simulink model "DualBuckPPS22016"  (R2024b)
settings: Solver=ode45  StartTime=0.0  StopTime=0.5  RelTol=1e-3
model workspace (MAT data in the model file):
  D = 50
  T = 0.0333333333333
undefined symbols (not defined in the file): D_T_DOWN_Given, D_T_UP_Given, DiscIntNeverNeededParam, P, T_pulse, TP
libraries: spsOnDelayLib x30, dspsnks4 x12, dspfdesign x11, spsCurrentMeasurementLib x11, spsSeriesRLCBranchLib x6, spsMosfetLib x4, slpidlib x4, spsVoltageMeasurementLib x4, simulink x3, spsControlledCurrentSourceLib x1, spsDCVoltageSourceLib x1, spspowerguiLib x1
(part 2 of 2)

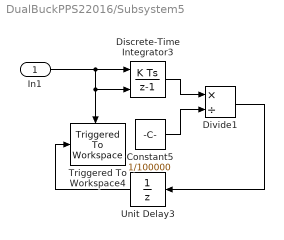
== system DualBuckPPS22016/Subsystem5 ==
  In1 : Inport
  Constant5 : Constant  Value=1/100000
  Discrete-Time Integrator3 : DiscreteIntegrator  ExternalReset=falling  SampleTime=-1  ICPrevOutput=DiscIntNeverNeededParam  ICPrevScaledInput=DiscIntNeverNeededParam
  Divide1 : Product  Inputs=*/
  Triggered To Workspace4 : dspsnks4/Triggered To Workspace  TriggerType=Falling edge  VariableName=PWM_S_DOWN  Buffer=1000  Save2DMode=2-D array (concatenate along first dimension)
      settings: FixptAsFi=off
  Unit Delay3 : UnitDelay  SampleTime=-1  HasFrameUpgradeWarning=on
  wires:
  Unit Delay3/1 -> Triggered To Workspace4/1
  Discrete-Time Integrator3/1 -> Divide1/1
  Constant5/1 -> Divide1/2
  Divide1/1 -> Unit Delay3/1
  In1/1 -> Discrete-Time Integrator3/1, Triggered To Workspace4/Trigger, Discrete-Time Integrator3/2

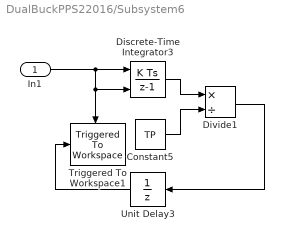
== system DualBuckPPS22016/Subsystem6 ==
  In1 : Inport
  Constant5 : Constant  Value=TP
  Discrete-Time Integrator3 : DiscreteIntegrator  ExternalReset=falling  SampleTime=-1  ICPrevOutput=DiscIntNeverNeededParam  ICPrevScaledInput=DiscIntNeverNeededParam
  Divide1 : Product  Inputs=*/
  Triggered To Workspace1 : dspsnks4/Triggered To Workspace  TriggerType=Falling edge  VariableName=VC1_DOWN  Buffer=1000  Save2DMode=2-D array (concatenate along first dimension)
      settings: FixptAsFi=off
  Unit Delay3 : UnitDelay  SampleTime=-1  HasFrameUpgradeWarning=on
  wires:
  Unit Delay3/1 -> Triggered To Workspace1/1
  Discrete-Time Integrator3/1 -> Divide1/1
  In1/1 -> Discrete-Time Integrator3/1, Discrete-Time Integrator3/2, Triggered To Workspace1/Trigger
  Constant5/1 -> Divide1/2
  Divide1/1 -> Unit Delay3/1

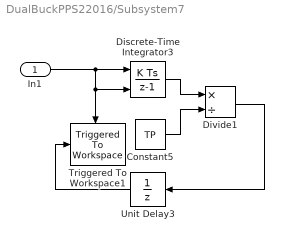
== system DualBuckPPS22016/Subsystem7 ==
  In1 : Inport
  Constant5 : Constant  Value=TP
  Discrete-Time Integrator3 : DiscreteIntegrator  ExternalReset=falling  SampleTime=-1  ICPrevOutput=DiscIntNeverNeededParam  ICPrevScaledInput=DiscIntNeverNeededParam
  Divide1 : Product  Inputs=*/
  Triggered To Workspace1 : dspsnks4/Triggered To Workspace  TriggerType=Falling edge  VariableName=VG1_UP  Buffer=1000  Save2DMode=2-D array (concatenate along first dimension)
      settings: FixptAsFi=off
  Unit Delay3 : UnitDelay  SampleTime=-1  HasFrameUpgradeWarning=on
  wires:
  Unit Delay3/1 -> Triggered To Workspace1/1
  Discrete-Time Integrator3/1 -> Divide1/1
  In1/1 -> Discrete-Time Integrator3/1, Discrete-Time Integrator3/2, Triggered To Workspace1/Trigger
  Constant5/1 -> Divide1/2
  Divide1/1 -> Unit Delay3/1

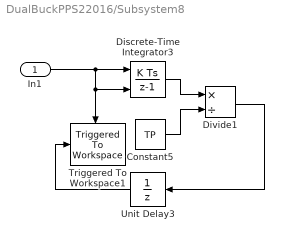
== system DualBuckPPS22016/Subsystem8 ==
  In1 : Inport
  Constant5 : Constant  Value=TP
  Discrete-Time Integrator3 : DiscreteIntegrator  ExternalReset=falling  SampleTime=-1  ICPrevOutput=DiscIntNeverNeededParam  ICPrevScaledInput=DiscIntNeverNeededParam
  Divide1 : Product  Inputs=*/
  Triggered To Workspace1 : dspsnks4/Triggered To Workspace  TriggerType=Falling edge  VariableName=VG1_DOWN  Buffer=1000  Save2DMode=2-D array (concatenate along first dimension)
      settings: FixptAsFi=off
  Unit Delay3 : UnitDelay  SampleTime=-1  HasFrameUpgradeWarning=on
  wires:
  Divide1/1 -> Unit Delay3/1
  Constant5/1 -> Divide1/2
  In1/1 -> Triggered To Workspace1/Trigger, Discrete-Time Integrator3/2, Discrete-Time Integrator3/1
  Discrete-Time Integrator3/1 -> Divide1/1
  Unit Delay3/1 -> Triggered To Workspace1/1

== system DualBuckPPS22016/Subsystem9 ==
  In : Inport
  On Delay10 : spsOnDelayLib/On Delay  DelayType=On delay  delay=10e-6  ic=0  Ts=0
  On Delay11 : spsOnDelayLib/On Delay  DelayType=Off delay  delay=ceil(TP*1e5)*1e-5-TP  ic=0  Ts=0
  Out : Outport
  wires:
  On Delay10/1 -> On Delay11/1
  In/1 -> On Delay10/1
  On Delay11/1 -> Out/1

== system DualBuckPPS22016/Triggered Subsystem ==
  In1 : Inport
  Trigger : TriggerPort  VariantControl=(inherit)
  Out1 : Outport
  wires:
  In1/1 -> Out1/1

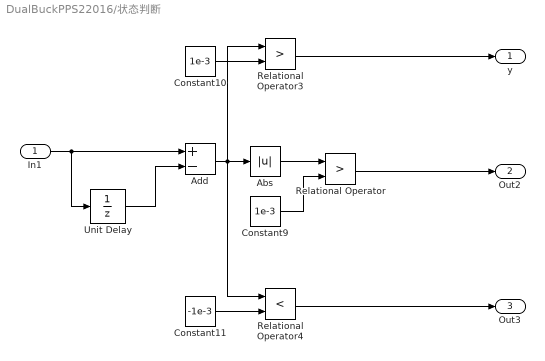
== system DualBuckPPS22016/状态判断 ==
  In1 : Inport
  Abs : Abs  SaturateOnIntegerOverflow=off
  Add : Sum  Inputs=+-
  Constant10 : Constant  Value=1e-3
  Constant11 : Constant  Value=-1e-3
  Constant9 : Constant  Value=1e-3
  Relational Operator : RelationalOperator  Operator=>  OutDataTypeStr=boolean  RndMeth=Simplest  InputSameDT=off
  Relational Operator3 : RelationalOperator  Operator=>  OutDataTypeStr=boolean  RndMeth=Simplest  InputSameDT=off
  Relational Operator4 : RelationalOperator  Operator=<  OutDataTypeStr=boolean  RndMeth=Simplest  InputSameDT=off
  Unit Delay : UnitDelay  SampleTime=-1  HasFrameUpgradeWarning=on
  y : Outport
  Out2 : Outport  Port=2
  Out3 : Outport  Port=3
  wires:
  In1/1 -> Unit Delay/1, Add/1
  Constant10/1 -> Relational Operator3/2
  Unit Delay/1 -> Add/2
  Constant9/1 -> Relational Operator/2
  Constant11/1 -> Relational Operator4/2
  Add/1 -> Relational Operator4/1, Relational Operator3/1, Abs/1
  Abs/1 -> Relational Operator/1
  Relational Operator3/1 -> y/1
  Relational Operator/1 -> Out2/1
  Relational Operator4/1 -> Out3/1

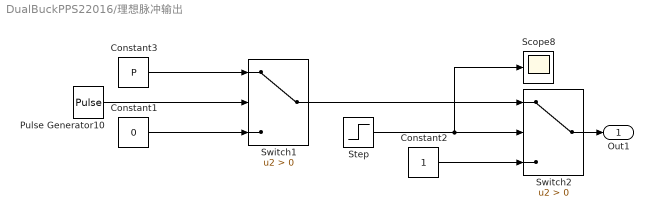
== system DualBuckPPS22016/理想脉冲输出 ==
  Constant1 : Constant  Value=0
  Constant2 : Constant
  Constant3 : Constant  Value=P
  Pulse Generator10 : DiscretePulseGenerator  PulseType=Time based  Period=T  PulseWidth=D  VectorParams1D=off
  Scope8 : Scope
  Step : Step  Time=0  SampleTime=0
  Switch1 : Switch  Criteria=u2 > Threshold  SaturateOnIntegerOverflow=off  InputSameDT=off
  Switch2 : Switch  Criteria=u2 > Threshold  SaturateOnIntegerOverflow=off  InputSameDT=off
  Out1 : Outport
  wires:
  Switch2/1 -> Out1/1
  Constant1/1 -> Switch1/3
  Step/1 -> Scope8/1, Switch2/2
  Switch1/1 -> Switch2/1
  Pulse Generator10/1 -> Switch1/2
  Constant2/1 -> Switch2/3
  Constant3/1 -> Switch1/1

== matlab function DualBuckPPS22016/MATLAB Function4 ==
  data: Q_main output; Q_sync output; Vref input; Vo input; Iref_ext input; iL input; voltage_PI_out output; current_error output; T_period output
function [Q_main, Q_sync, voltage_PI_out, ...
          current_error, T_period] = ...
    Buck_Double_COT(Vref, Vo, Iref_ext, iL)
%#codegen
%
% 单路同步Buck：
% 电压外环PI + 电流比较型COT控制
%
% 输入：
% Vref     ：输出电压参考值
% Vo       ：实际输出电压
% Iref_ext ：外部电感电流参考值
% iL       ：实际电感电流
%
% 输出：
% Q_main         ：主开关驱动信号
% Q_sync         ：同步开关驱动信号
% voltage_PI_out ：电压外环PI输出
% current_error  ：电流比较误差
% T_period       ：最近一个完整COT开关周期，单位为s
%
% 电流误差保持原有定义：
%
% current_error = voltage_PI_out - Iref_ext - iL
%
% 当current_error >= I_trigger，
% 并且满足最小关断时间时，
% 主开关固定导通Ton。

%% ===================== 1. 控制参数 =====================

Ts = 100e-9;                       % MATLAB Function执行周期

Kpv = 0.02;                        % 电压外环比例系数

Kiv = 0.2;                         % 电压外环积分系数

Ton = 2e-6;                        % COT固定导通时间

Toff_min = Ts;                     % 两个脉冲之间的最小关断时间

I_trigger = 0.2;                   % COT电流误差触发阈值

N_on = max(1, round(Ton / Ts));    % 固定导通时间对应的采样点数

N_off = max(1, round(Toff_min / Ts));
                                      % 最小关断时间对应的采样点数

%% ===================== 2. 持久变量 =====================

persistent voltage_integral        % 电压PI积分项

persistent on_count                % 固定导通剩余采样点数

persistent off_count               % 当前连续关断采样点数

persistent period_count            % 当前开关周期采样点计数

persistent last_period_count       % 最近一个完整开关周期采样点数

persistent first_pulse_generated   % 是否已经产生过第一个脉冲

%% ===================== 3. 第一次运行初始化 =====================

if isempty(voltage_integral)

    voltage_integral = 0.0;         % PI积分项初始化

    on_count = 0.0;                 % 初始不处于固定导通阶段

    off_count = N_off;              % 初始允许产生第一个脉冲

    period_count = 0.0;             % 当前周期计数初始化

    last_period_count = 0.0;        % 尚未测得完整周期

    first_pulse_generated = false;  % 尚未产生第一个脉冲

end

%% ===================== 4. 电压外环PI =====================

voltage_error = Vref - Vo;          % 计算输出电压误差

voltage_integral = voltage_integral ...
                 + Kiv * voltage_error * Ts;
                                      % 更新电压PI积分项

voltage_PI_out = Kpv * voltage_error ...
               + voltage_integral;
                                      % 计算电压PI输出

%% ===================== 5. 电流比较与触发请求 =====================

current_error = voltage_PI_out ...
              - Iref_ext ...
              - iL;
                                      % 保持原有电流误差逻辑

cot_request = current_error >= I_trigger;
                                      % 判断是否满足COT触发条件

%% ===================== 6. 开关周期计数 =====================

period_count = period_count + 1.0;  % 统计两次脉冲起点之间的采样点数

%% ===================== 7. 默认主开关状态 =====================

Q_main = false;                     % 默认主开关关断

%% ===================== 8. COT固定导通阶段 =====================

if on_count > 0.0

    Q_main = true;                  % 固定导通时间内保持主开关导通

    on_count = on_count - 1.0;      % 固定导通剩余计数减1

    if on_count <= 0.0

        on_count = 0.0;             % 固定导通时间结束

        off_count = 0.0;            % 开始统计最小关断时间

    end

%% ===================== 9. COT关断等待阶段 =====================

else

    if cot_request && (off_count >= N_off)

        % 第一次脉冲没有前一个脉冲，因此不能计算完整周期
        if first_pulse_generated

            last_period_count = max(1.0, period_count);
                                      % 保存本次脉冲与上次脉冲之间的周期

        else

            first_pulse_generated = true;
                                      % 标记第一个脉冲已经产生

        end

        period_count = 0.0;         % 从当前脉冲起点重新计算周期

        Q_main = true;              % 当前采样点立即导通主开关

        on_count = N_on - 1.0;      % 当前点已占用一个导通采样点

        off_count = 0.0;            % 清零关断时间计数

    else

        off_count = off_count + 1.0;
                                      % 未触发时继续累计关断时间

    end

end

%% ===================== 10. 同步开关输出 =====================

Q_sync = ~Q_main;                   % 不设置死区，上下管直接互补

%% ===================== 11. 实际COT周期输出 =====================

T_period = last_period_count * Ts;  % 计算最近一个完整COT周期，单位为s

end

== matlab function DualBuckPPS22016/MATLAB Function5 ==
  data: Q_main output; Q_sync output; Vref input; Vo input; Iref_ext input; iL input; voltage_PI_out output; current_error output; T_period output
function [Q_main, Q_sync, voltage_PI_out, ...
          current_error, T_period] = ...
    Buck_Double_COT(Vref, Vo, Iref_ext, iL)
%#codegen
%
% 单路同步Buck：
% 电压外环PI + 电流比较型COT控制
%
% 输入：
% Vref     ：输出电压参考值
% Vo       ：实际输出电压
% Iref_ext ：外部电感电流参考值
% iL       ：实际电感电流
%
% 输出：
% Q_main         ：主开关驱动信号
% Q_sync         ：同步开关驱动信号
% voltage_PI_out ：电压外环PI输出
% current_error  ：电流比较误差
% T_period       ：最近一个完整COT开关周期，单位为s
%
% 电流误差保持原有定义：
%
% current_error = voltage_PI_out - Iref_ext - iL
%
% 当current_error >= I_trigger，
% 并且满足最小关断时间时，
% 主开关固定导通Ton。

%% ===================== 1. 控制参数 =====================

Ts = 100e-9;                       % MATLAB Function执行周期

Kpv = 0.02;                        % 电压外环比例系数

Kiv = 0.2;                         % 电压外环积分系数

Ton = 2e-6;                        % COT固定导通时间

Toff_min = Ts;                     % 两个脉冲之间的最小关断时间

I_trigger = 0.2;                   % COT电流误差触发阈值

N_on = max(1, round(Ton / Ts));    % 固定导通时间对应的采样点数

N_off = max(1, round(Toff_min / Ts));
                                      % 最小关断时间对应的采样点数

%% ===================== 2. 持久变量 =====================

persistent voltage_integral        % 电压PI积分项

persistent on_count                % 固定导通剩余采样点数

persistent off_count               % 当前连续关断采样点数

persistent period_count            % 当前开关周期采样点计数

persistent last_period_count       % 最近一个完整开关周期采样点数

persistent first_pulse_generated   % 是否已经产生过第一个脉冲

%% ===================== 3. 第一次运行初始化 =====================

if isempty(voltage_integral)

    voltage_integral = 0.0;         % PI积分项初始化

    on_count = 0.0;                 % 初始不处于固定导通阶段

    off_count = N_off;              % 初始允许产生第一个脉冲

    period_count = 0.0;             % 当前周期计数初始化

    last_period_count = 0.0;        % 尚未测得完整周期

    first_pulse_generated = false;  % 尚未产生第一个脉冲

end

%% ===================== 4. 电压外环PI =====================

voltage_error = Vref - Vo;          % 计算输出电压误差

voltage_integral = voltage_integral ...
                 + Kiv * voltage_error * Ts;
                                      % 更新电压PI积分项

voltage_PI_out = Kpv * voltage_error ...
               + voltage_integral;
                                      % 计算电压PI输出

%% ===================== 5. 电流比较与触发请求 =====================

current_error = voltage_PI_out ...
              - Iref_ext ...
              - iL;
                                      % 保持原有电流误差逻辑

cot_request = current_error >= I_trigger;
                                      % 判断是否满足COT触发条件

%% ===================== 6. 开关周期计数 =====================

period_count = period_count + 1.0;  % 统计两次脉冲起点之间的采样点数

%% ===================== 7. 默认主开关状态 =====================

Q_main = false;                     % 默认主开关关断

%% ===================== 8. COT固定导通阶段 =====================

if on_count > 0.0

    Q_main = true;                  % 固定导通时间内保持主开关导通

    on_count = on_count - 1.0;      % 固定导通剩余计数减1

    if on_count <= 0.0

        on_count = 0.0;             % 固定导通时间结束

        off_count = 0.0;            % 开始统计最小关断时间

    end

%% ===================== 9. COT关断等待阶段 =====================

else

    if cot_request && (off_count >= N_off)

        % 第一次脉冲没有前一个脉冲，因此不能计算完整周期
        if first_pulse_generated

            last_period_count = max(1.0, period_count);
                                      % 保存本次脉冲与上次脉冲之间的周期

        else

            first_pulse_generated = true;
                                      % 标记第一个脉冲已经产生

        end

        period_count = 0.0;         % 从当前脉冲起点重新计算周期

        Q_main = true;              % 当前采样点立即导通主开关

        on_count = N_on - 1.0;      % 当前点已占用一个导通采样点

        off_count = 0.0;            % 清零关断时间计数

    else

        off_count = off_count + 1.0;
                                      % 未触发时继续累计关断时间

    end

end

%% ===================== 10. 同步开关输出 =====================

Q_sync = ~Q_main;                   % 不设置死区，上下管直接互补

%% ===================== 11. 实际COT周期输出 =====================

T_period = last_period_count * Ts;  % 计算最近一个完整COT周期，单位为s

end

== matlab function DualBuckPPS22016/MATLAB Function6 ==
  settings: updateMethod=DISCRETE
  data: Flag input; PWM_gated output; PWM input; Total_on_time output; Flag_on_time output; Pre_on_time output; Post_on_time output; Done output
function [PWM_gated, Total_on_time, Flag_on_time, ...
          Pre_on_time, Post_on_time, Done] = ...
    PWM_Flag_Analyzer(Flag, PWM)
%#codegen
%
% 功能：
% 1. 对Flag和PWM执行逻辑与运算；
% 2. 统计Flag=1区间内PWM的导通时间；
% 3. 若Flag开始时PWM已经导通，向前补齐该PWM脉冲；
% 4. 若Flag结束时PWM仍然导通，继续统计到PWM关断；
% 5. 计算前补偿、区间内、后补偿及总导通时间；
% 6. 仅在0.05 s～0.45 s内执行统计。
%
% 输入：
% Flag：标志位，大于0.5认为是逻辑1
% PWM ：PWM信号，大于0.5认为是逻辑1
%
% 输出：
% PWM_gated     ：Flag与PWM相与后的信号
% Total_on_time ：完整补偿后的PWM总导通时间，单位s
% Flag_on_time  ：Flag=1区间内PWM导通时间，单位s
% Pre_on_time   ：Flag上升沿之前的PWM补偿时间，单位s
% Post_on_time  ：Flag下降沿之后的PWM补偿时间，单位s
% Done          ：本次统计完成时输出一个采样周期的1

%% ===================== 1. 参数设置 =====================

Ts = 100e-9;                       % MATLAB Function实际执行周期

T_start = 0.05;                    % 模块开始统计的仿真时间

T_stop = 0.45;                     % 模块停止统计的仿真时间

%% ===================== 2. 持久变量 =====================

persistent sample_count            % MATLAB Function执行次数

persistent previous_flag           % 上一个采样时刻的Flag状态

persistent pwm_high_count          % 当前PWM连续高电平的采样点数

persistent state                   % 统计状态

persistent pre_count               % 前补偿PWM导通采样点数

persistent flag_count              % Flag区间PWM导通采样点数

persistent post_count              % 后补偿PWM导通采样点数

%% ===================== 3. 第一次运行初始化 =====================

if isempty(sample_count)

    sample_count = 0.0;             % 从仿真时间0开始计数

    previous_flag = false;          % 上一时刻Flag初始化为0

    pwm_high_count = 0.0;           % PWM连续高电平计数初始化为0

    state = uint8(0);               % 状态0表示等待Flag上升沿

    pre_count = 0.0;                % 前补偿计数初始化为0

    flag_count = 0.0;               % Flag区间计数初始化为0

    post_count = 0.0;               % 后补偿计数初始化为0

end

%% ===================== 4. 信号逻辑化 =====================

flag_now = Flag > 0.5;             % 将Flag转换为逻辑信号

pwm_now = PWM > 0.5;               % 将PWM转换为逻辑信号

current_time = sample_count * Ts;   % 根据采样次数计算当前仿真时间

%% ===================== 5. 默认输出 =====================

PWM_gated = 0.0;                    % 默认相与后的PWM为0

Done = 0.0;                         % 默认没有完成统计

Pre_on_time = pre_count * Ts;       % 当前前补偿时间

Flag_on_time = flag_count * Ts;     % 当前Flag区间导通时间

Post_on_time = post_count * Ts;     % 当前后补偿时间

Total_on_time = Pre_on_time ...
              + Flag_on_time ...
              + Post_on_time;       % 当前总导通时间

%% ===================== 6. 0.05 s以前不统计 =====================

if current_time < T_start

    previous_flag = false;          % 清除Flag历史状态

    pwm_high_count = 0.0;           % 不记录0.05 s以前的PWM历史

    state = uint8(0);               % 保持等待状态

    pre_count = 0.0;                % 清除前补偿计数

    flag_count = 0.0;               % 清除Flag区间计数

    post_count = 0.0;               % 清除后补偿计数

    PWM_gated = 0.0;                % 输出相与信号为0

    Total_on_time = 0.0;            % 输出总时间为0

    Flag_on_time = 0.0;             % 输出区间时间为0

    Pre_on_time = 0.0;              % 输出前补偿时间为0

    Post_on_time = 0.0;             % 输出后补偿时间为0

    Done = 0.0;                     % 完成标志为0

    sample_count = sample_count + 1.0;
                                      % 更新时间计数

    return;                          % 结束当前采样点计算

end

%% ===================== 7. 0.45 s以后停止统计 =====================

if current_time > T_stop

    PWM_gated = 0.0;                % 统计窗口外相与PWM输出为0

    Pre_on_time = pre_count * Ts;   % 保持最近的前补偿结果

    Flag_on_time = flag_count * Ts; % 保持最近的区间结果

    Post_on_time = post_count * Ts; % 保持最近的后补偿结果

    Total_on_time = Pre_on_time ...
                  + Flag_on_time ...
                  + Post_on_time;   % 保持最近的总导通时间

    Done = 0.0;                     % 停止时间后不产生完成脉冲

    sample_count = sample_count + 1.0;
                                      % 继续更新时间计数

    return;                          % 结束当前采样点计算

end

%% ===================== 8. Flag与PWM逻辑与 =====================

PWM_gated = double(flag_now && pwm_now);
                                      % 只保留Flag=1区间内的PWM波形

%% ===================== 9. Flag边沿检测 =====================

flag_rising = flag_now && ~previous_flag;
                                      % 检测Flag的上升沿

%% ===================== 10. 状态0：等待Flag上升沿 =====================

if state == uint8(0)

    if flag_rising

        pre_count = 0.0;             % 新区间开始时清除前补偿

        flag_count = 0.0;            % 清除Flag区间计数

        post_count = 0.0;            % 清除后补偿计数

        if pwm_now

            pre_count = pwm_high_count;
                                      % PWM已经导通时补偿上升沿前的部分

            flag_count = 1.0;        % 当前采样点属于Flag区间

        end

        state = uint8(1);            % 进入Flag=1区间统计状态

    end

%% ===================== 11. 状态1：统计Flag区间 =====================

elseif state == uint8(1)

    if flag_now

        if pwm_now

            flag_count = flag_count + 1.0;
                                      % Flag=1且PWM=1时累计导通时间

        end

    else

        if pwm_now

            post_count = 1.0;        % 当前点属于Flag结束后的PWM部分

            state = uint8(2);        % 进入后补偿状态

        else

            state = uint8(0);        % PWM已关断，本次统计完成

            Done = 1.0;              % 输出一个采样周期的完成脉冲

        end

    end

%% ===================== 12. 状态2：统计后补偿 =====================

elseif state == uint8(2)

    if pwm_now

        post_count = post_count + 1.0;
                                      % PWM仍导通，继续累计后补偿

    else

        state = uint8(0);            % PWM关断，返回等待状态

        Done = 1.0;                  % 本次统计完成

    end

%% ===================== 13. 异常状态恢复 =====================

else

    state = uint8(0);                % 恢复到等待状态

    pre_count = 0.0;                 % 清除前补偿计数

    flag_count = 0.0;                % 清除Flag区间计数

    post_count = 0.0;                % 清除后补偿计数

    Done = 0.0;                      % 不产生完成信号

end

%% ===================== 14. 更新时间输出 =====================

Pre_on_time = pre_count * Ts;       % 前补偿导通时间

Flag_on_time = flag_count * Ts;     % Flag区间PWM导通时间

Post_on_time = post_count * Ts;     % 后补偿PWM导通时间

Total_on_time = Pre_on_time ...
              + Flag_on_time ...
              + Post_on_time;       % 补偿后的PWM总导通时间

%% ===================== 15. 更新PWM连续高电平历史 =====================

if pwm_now

    pwm_high_count = pwm_high_count + 1.0;
                                      % PWM为高时累计连续导通点数

else

    pwm_high_count = 0.0;            % PWM关断时重新开始计数

end

%% ===================== 16. 更新Flag历史及时间 =====================

previous_flag = flag_now;           % 保存本次Flag供下一次边沿检测

sample_count = sample_count + 1.0;  % 当前仿真时间增加一个采样周期

end

== matlab function DualBuckPPS22016/MATLAB Function7 ==
  settings: updateMethod=DISCRETE
  data: Flag input; PWM_gated output; PWM input; Total_on_time output; Flag_on_time output; Pre_on_time output; Post_on_time output; Done output
function [PWM_gated, Total_on_time, Flag_on_time, ...
          Pre_on_time, Post_on_time, Done] = ...
    PWM_Flag_Analyzer(Flag, PWM)
%#codegen
%
% 功能：
% 1. 对Flag和PWM执行逻辑与运算；
% 2. 统计Flag=1区间内PWM的导通时间；
% 3. 若Flag开始时PWM已经导通，向前补齐该PWM脉冲；
% 4. 若Flag结束时PWM仍然导通，继续统计到PWM关断；
% 5. 计算前补偿、区间内、后补偿及总导通时间；
% 6. 仅在0.05 s～0.45 s内执行统计。
%
% 输入：
% Flag：标志位，大于0.5认为是逻辑1
% PWM ：PWM信号，大于0.5认为是逻辑1
%
% 输出：
% PWM_gated     ：Flag与PWM相与后的信号
% Total_on_time ：完整补偿后的PWM总导通时间，单位s
% Flag_on_time  ：Flag=1区间内PWM导通时间，单位s
% Pre_on_time   ：Flag上升沿之前的PWM补偿时间，单位s
% Post_on_time  ：Flag下降沿之后的PWM补偿时间，单位s
% Done          ：本次统计完成时输出一个采样周期的1

%% ===================== 1. 参数设置 =====================

Ts = 100e-9;                       % MATLAB Function实际执行周期

T_start = 0.05;                    % 模块开始统计的仿真时间

T_stop = 0.45;                     % 模块停止统计的仿真时间

%% ===================== 2. 持久变量 =====================

persistent sample_count            % MATLAB Function执行次数

persistent previous_flag           % 上一个采样时刻的Flag状态

persistent pwm_high_count          % 当前PWM连续高电平的采样点数

persistent state                   % 统计状态

persistent pre_count               % 前补偿PWM导通采样点数

persistent flag_count              % Flag区间PWM导通采样点数

persistent post_count              % 后补偿PWM导通采样点数

%% ===================== 3. 第一次运行初始化 =====================

if isempty(sample_count)

    sample_count = 0.0;             % 从仿真时间0开始计数

    previous_flag = false;          % 上一时刻Flag初始化为0

    pwm_high_count = 0.0;           % PWM连续高电平计数初始化为0

    state = uint8(0);               % 状态0表示等待Flag上升沿

    pre_count = 0.0;                % 前补偿计数初始化为0

    flag_count = 0.0;               % Flag区间计数初始化为0

    post_count = 0.0;               % 后补偿计数初始化为0

end

%% ===================== 4. 信号逻辑化 =====================

flag_now = Flag > 0.5;             % 将Flag转换为逻辑信号

pwm_now = PWM > 0.5;               % 将PWM转换为逻辑信号

current_time = sample_count * Ts;   % 根据采样次数计算当前仿真时间

%% ===================== 5. 默认输出 =====================

PWM_gated = 0.0;                    % 默认相与后的PWM为0

Done = 0.0;                         % 默认没有完成统计

Pre_on_time = pre_count * Ts;       % 当前前补偿时间

Flag_on_time = flag_count * Ts;     % 当前Flag区间导通时间

Post_on_time = post_count * Ts;     % 当前后补偿时间

Total_on_time = Pre_on_time ...
              + Flag_on_time ...
              + Post_on_time;       % 当前总导通时间

%% ===================== 6. 0.05 s以前不统计 =====================

if current_time < T_start

    previous_flag = false;          % 清除Flag历史状态

    pwm_high_count = 0.0;           % 不记录0.05 s以前的PWM历史

    state = uint8(0);               % 保持等待状态

    pre_count = 0.0;                % 清除前补偿计数

    flag_count = 0.0;               % 清除Flag区间计数

    post_count = 0.0;               % 清除后补偿计数

    PWM_gated = 0.0;                % 输出相与信号为0

    Total_on_time = 0.0;            % 输出总时间为0

    Flag_on_time = 0.0;             % 输出区间时间为0

    Pre_on_time = 0.0;              % 输出前补偿时间为0

    Post_on_time = 0.0;             % 输出后补偿时间为0

    Done = 0.0;                     % 完成标志为0

    sample_count = sample_count + 1.0;
                                      % 更新时间计数

    return;                          % 结束当前采样点计算

end

%% ===================== 7. 0.45 s以后停止统计 =====================

if current_time > T_stop

    PWM_gated = 0.0;                % 统计窗口外相与PWM输出为0

    Pre_on_time = pre_count * Ts;   % 保持最近的前补偿结果

    Flag_on_time = flag_count * Ts; % 保持最近的区间结果

    Post_on_time = post_count * Ts; % 保持最近的后补偿结果

    Total_on_time = Pre_on_time ...
                  + Flag_on_time ...
                  + Post_on_time;   % 保持最近的总导通时间

    Done = 0.0;                     % 停止时间后不产生完成脉冲

    sample_count = sample_count + 1.0;
                                      % 继续更新时间计数

    return;                          % 结束当前采样点计算

end

%% ===================== 8. Flag与PWM逻辑与 =====================

PWM_gated = double(flag_now && pwm_now);
                                      % 只保留Flag=1区间内的PWM波形

%% ===================== 9. Flag边沿检测 =====================

flag_rising = flag_now && ~previous_flag;
                                      % 检测Flag的上升沿

%% ===================== 10. 状态0：等待Flag上升沿 =====================

if state == uint8(0)

    if flag_rising

        pre_count = 0.0;             % 新区间开始时清除前补偿

        flag_count = 0.0;            % 清除Flag区间计数

        post_count = 0.0;            % 清除后补偿计数

        if pwm_now

            pre_count = pwm_high_count;
                                      % PWM已经导通时补偿上升沿前的部分

            flag_count = 1.0;        % 当前采样点属于Flag区间

        end

        state = uint8(1);            % 进入Flag=1区间统计状态

    end

%% ===================== 11. 状态1：统计Flag区间 =====================

elseif state == uint8(1)

    if flag_now

        if pwm_now

            flag_count = flag_count + 1.0;
                                      % Flag=1且PWM=1时累计导通时间

        end

    else

        if pwm_now

            post_count = 1.0;        % 当前点属于Flag结束后的PWM部分

            state = uint8(2);        % 进入后补偿状态

        else

            state = uint8(0);        % PWM已关断，本次统计完成

            Done = 1.0;              % 输出一个采样周期的完成脉冲

        end

    end

%% ===================== 12. 状态2：统计后补偿 =====================

elseif state == uint8(2)

    if pwm_now

        post_count = post_count + 1.0;
                                      % PWM仍导通，继续累计后补偿

    else

        state = uint8(0);            % PWM关断，返回等待状态

        Done = 1.0;                  % 本次统计完成

    end

%% ===================== 13. 异常状态恢复 =====================

else

    state = uint8(0);                % 恢复到等待状态

    pre_count = 0.0;                 % 清除前补偿计数

    flag_count = 0.0;                % 清除Flag区间计数

    post_count = 0.0;                % 清除后补偿计数

    Done = 0.0;                      % 不产生完成信号

end

%% ===================== 14. 更新时间输出 =====================

Pre_on_time = pre_count * Ts;       % 前补偿导通时间

Flag_on_time = flag_count * Ts;     % Flag区间PWM导通时间

Post_on_time = post_count * Ts;     % 后补偿PWM导通时间

Total_on_time = Pre_on_time ...
              + Flag_on_time ...
              + Post_on_time;       % 补偿后的PWM总导通时间

%% ===================== 15. 更新PWM连续高电平历史 =====================

if pwm_now

    pwm_high_count = pwm_high_count + 1.0;
                                      % PWM为高时累计连续导通点数

else

    pwm_high_count = 0.0;            % PWM关断时重新开始计数

end

%% ===================== 16. 更新Flag历史及时间 =====================

previous_flag = flag_now;           % 保存本次Flag供下一次边沿检测

sample_count = sample_count + 1.0;  % 当前仿真时间增加一个采样周期

end
